simulink model "test_FAST_qLPVMPCflapIPC"  (R2023a)
settings: Solver=FixedStepAuto  StartTime=0.0  StopTime=OutTable.Time(end)  FixedStep=DT  RelTol=1e-3
values from neighbouring files (symbols this model uses):
  DT = 0.008    [initWorkspace.m]    (also in runCompareCtrl.m)
  ipcMaxRateCtrl = 13    [initWorkspace.m]
  ipcParCtrl = designMPC.ipcParCtrl    [initWorkspace.m]
  Lin_points : value not decoded    [DD_test.sldd]
undefined symbols (not defined in the file or in its folder): Rotor_Lambda
settings Model: DataDictionary=DD_test.sldd  ExtModeTrigMode=oneshot  Creator=Hazim Namik  LastModifiedBy=jdi
settings SolverCC: AlgebraicLoopSolver=TrustRegion  AutoInsertRateTranBlk=on
settings DataIOCC: LimitDataPoints=on  SaveFormat=Array  ReturnWorkspaceOutputs=off
settings OptimizationCC: BlockReduction=off  BooleanDataType=off  LifeSpan=inf
settings DebuggingCC: SaveWithParameterizedLinksMsg=none  UnderspecifiedInitializationDetection=Classic  MergeDetectMultiDrivingBlocksExec=none  SignalResolutionControl=TryResolveAllWithWarning  UnconnectedInputMsg=warning  UnconnectedOutputMsg=warning  UnconnectedLineMsg=warning  SFUnexpectedBacktrackingDiag=warning  SFNoUnconditionalDefaultTransitionDiag=warning  SFExecutionAtInitializationDiag=none  ArithmeticOperatorsInVariantConditions=warning
settings HardwareCC: ProdBitPerPointer=32  ProdBitPerSizeT=32  ProdBitPerPtrDiffT=32  ProdLargestAtomicFloat=None  ProdIntDivRoundTo=Undefined  ProdEndianess=Unspecified  ProdWordSize=32  ProdHWDeviceType=32-bit Generic  TargetUnknown=on
settings ModelReferenceCC: EnableRefExpFcnMdlSchedulingChecks=on  PropagateSignalLabelsOutOfModel=off
settings SFSimCC: SimUseLocalCustomCode=off  CustomCodeUndefinedFunction=UseInterfaceOnly
settings RTWCC: RTWUseLocalCustomCode=off  DLArmComputeVersion=19.05
settings CodeAppCC: StateflowObjectComments=on
settings GRTTargetCC: TargetLangStandard=C89/C90 (ANSI)
settings ConfigComp: CovMetricSettings=dw  CovSaveCumulativeToWorkspaceVar=on  CovSaveSingleToWorkspaceVar=on  CovExternalEMLEnable=off

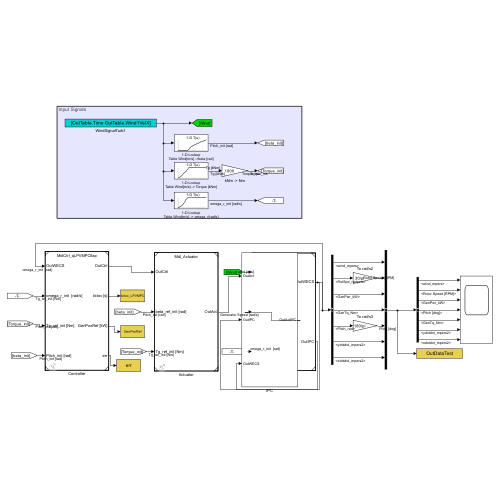
[thumbnail: Simulink's stored preview of the top-level diagram]
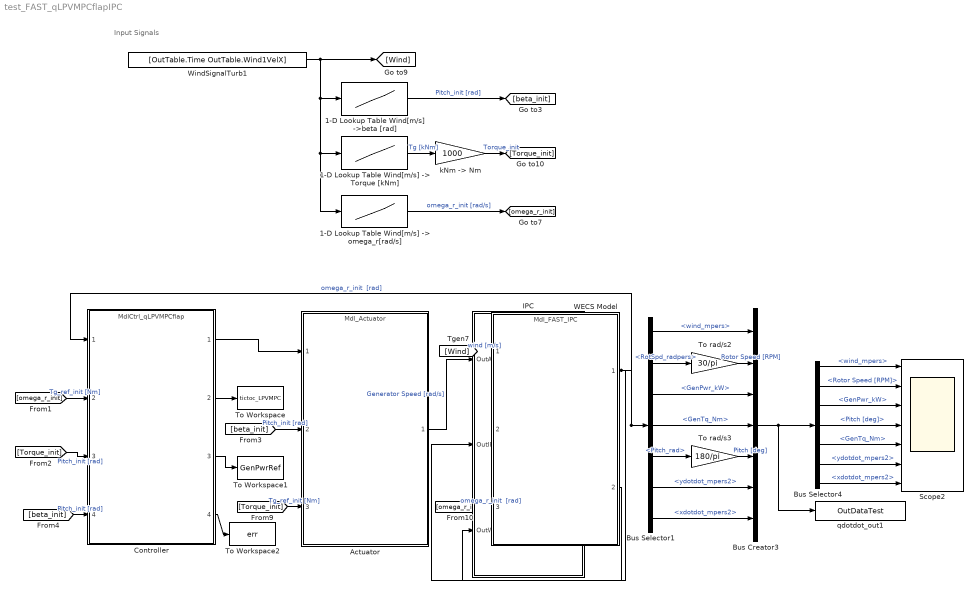
== system test_FAST_qLPVMPCflapIPC ==
  note: Input Signals
  "1-D Lookup Table Wind[m/s] -> Torque [kNm]" : Lookup_n-D  NumberOfTableDimensions=1  BreakpointsForDimension1=Lin_points.V  BreakpointsForDimension2=Rotor_Lambda  Table=Lin_points.Torque  InternalRulePriority=Speed  RndMeth=Simplest
  "1-D Lookup Table Wind[m/s] -> omega_r[rad/s]" : Lookup_n-D  NumberOfTableDimensions=1  BreakpointsForDimension1=Lin_points.V  BreakpointsForDimension2=Rotor_Lambda  Table=Lin_points.RSpeed  InternalRulePriority=Speed  RndMeth=Simplest
  1-D Lookup Table Wind[m/s] ->beta [rad] : Lookup_n-D  NumberOfTableDimensions=1  BreakpointsForDimension1=Lin_points.V  BreakpointsForDimension2=Rotor_Lambda  Table=Lin_points.Pitch  InternalRulePriority=Speed  RndMeth=Simplest
  Actuator : ModelReference  ModelNameDialog=Mdl_Actuator.slx  SimulationMode=Normal  ModelReferenceVersion=7.0
  Bus Creator3 : BusCreator  Inputs=7
  Bus Selector1 : BusSelector  OutputSignals=wind_mpers,RotSpd_radpers,GenPwr_kW,GenTq_Nm,Pitch_rad,ydotdot_mpers2,xdotdot_mpers2
  Bus Selector4 : BusSelector  OutputSignals=wind_mpers,Rotor Speed [RPM],GenPwr_kW,Pitch [deg],GenTq_Nm,ydotdot_mpers2,xdotdot_mpers2
  Controller : ModelReference  ModelNameDialog=MdlCtrl_qLPVMPCflap  SimulationMode=Normal  ModelReferenceVersion=7.57
  IPC : Subsystem
  Scope2 : Scope  NumInputPorts=7
      settings: Tag=Scope
  To Workspace : ToWorkspace  VariableName=tictoc_LPVMPC  SaveFormat=Timeseries  SampleTime=-1
  To Workspace1 : ToWorkspace  VariableName=GenPwrRef  SaveFormat=Timeseries  SampleTime=-1
  To Workspace2 : ToWorkspace  VariableName=err  SaveFormat=Timeseries  SampleTime=-1
  To rad/s2 : Gain  Gain=30/pi
  To rad/s3 : Gain  Gain=180/pi
  WECS Model : ModelReference  ModelNameDialog=Mdl_FAST_IPC  SimulationMode=Normal  ModelReferenceVersion=8.1
  WindSignalTurb1 : FromWorkspace  VariableName=[OutTable.Time OutTable.Wind1VelX]  SampleTime=DT  OutputAfterFinalValue=Holding final value
  "kNm -> Nm" : Gain  Gain=1000
  qdotdot_out1 : ToWorkspace  VariableName=OutDataTest  SampleTime=-1
  wires:
  [Torque_init] -> Controller/3  "Pitch_init [rad]"
  WindSignalTurb1/1 -> [Wind], "1-D Lookup Table Wind[m/s] -> omega_r[rad/s]"/1, "1-D Lookup Table Wind[m/s] -> Torque [kNm]"/1, 1-D Lookup Table Wind[m/s] ->beta [rad]/1
  "kNm -> Nm"/1 -> [Torque_init]  "Torque_init"
  [omega_r_init] -> Controller/2  "Tg_ref_init [Nm]"
  "1-D Lookup Table Wind[m/s] -> omega_r[rad/s]"/1 -> [omega_r_init]  "omega_r_init [rad/s]"
  [Wind] -> WECS Model/1  "wind [m/s]"
  1-D Lookup Table Wind[m/s] ->beta [rad]/1 -> [beta_init]  "Pitch_init [rad]"
  "1-D Lookup Table Wind[m/s] -> Torque [kNm]"/1 -> "kNm -> Nm"/1  "Tg [kNm]"
  [Torque_init] -> Actuator/3  "Tg_ref_init [Nm]"
  [omega_r_init] -> WECS Model/3  "omega_r_init  [rad]"
  Controller/3 -> To Workspace1/1
  [beta_init] -> Actuator/2  "Pitch_init [rad]"
  Bus Selector1/5 -> To rad/s3/1  "<Pitch_rad>"
  To rad/s2/1 -> Bus Creator3/2  "Rotor Speed [RPM]"
  Bus Creator3/1 -> Bus Selector4/1, qdotdot_out1/1
  Bus Selector4/4 -> Scope2/4  "<Pitch [deg]>"
  Bus Selector4/7 -> Scope2/7  "<xdotdot_mpers2>"
  Bus Selector4/6 -> Scope2/6  "<ydotdot_mpers2>"
  Bus Selector4/1 -> Scope2/1  "<wind_mpers>"
  To rad/s3/1 -> Bus Creator3/5  "Pitch [deg]"
  Bus Selector4/5 -> Scope2/5  "<GenTq_Nm>"
  Bus Selector1/2 -> To rad/s2/1  "<RotSpd_radpers>"
  Bus Selector1/1 -> Bus Creator3/1  "<wind_mpers>"
  Bus Selector1/4 -> Bus Creator3/4  "<GenTq_Nm>"
  Bus Selector1/3 -> Bus Creator3/3  "<GenPwr_kW>"
  Bus Selector1/7 -> Bus Creator3/7  "<xdotdot_mpers2>"
  Bus Selector1/6 -> Bus Creator3/6  "<ydotdot_mpers2>"
  Bus Selector4/3 -> Scope2/3  "<GenPwr_kW>"
  Bus Selector4/2 -> Scope2/2  "<Rotor Speed [RPM]>"
  WECS Model/1 -> Bus Selector1/1, Controller/1, IPC/3(OutWECS)  "omega_r_init  [rad]"
  [beta_init] -> Controller/4  "Pitch_init [rad]"
  Controller/1 -> Actuator/1
  Controller/2 -> To Workspace/1
  Controller/4 -> To Workspace2/1
  Actuator/1 -> IPC/1(OutAct)  "Generator Speed [rad/s]"
  WECS Model/2 -> IPC/2(OutIPC)
  IPC/1(OutActIPC) -> WECS Model/2

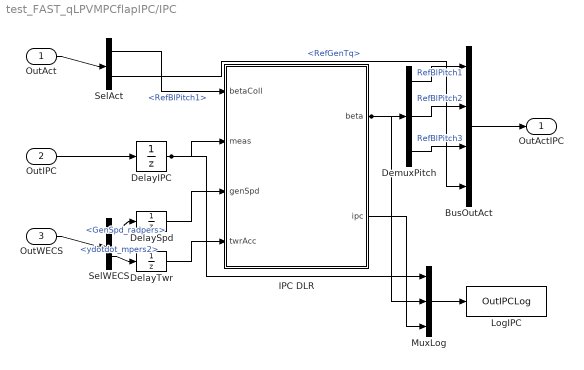
== system test_FAST_qLPVMPCflapIPC/IPC ==
  OutAct : Inport
  OutIPC : Inport  Port=2
  OutWECS : Inport  Port=3
  BusOutAct : BusCreator  Inputs=4
  DelayIPC : UnitDelay  InitialCondition=[0 0 0 0]  SampleTime=DT  HasFrameUpgradeWarning=on
  DelaySpd : UnitDelay  SampleTime=DT  HasFrameUpgradeWarning=on
  DelayTwr : UnitDelay  SampleTime=DT  HasFrameUpgradeWarning=on
  DemuxPitch : Demux  Outputs=3
  IPC DLR : MATLAB Function  TreatAsAtomicUnit=on
  LogIPC : ToWorkspace  VariableName=OutIPCLog  SampleTime=DT
  MuxLog : Mux  Inputs=3
  SelAct : BusSelector  OutputSignals=RefBlPitch1,RefGenTq
  SelWECS : BusSelector  OutputSignals=GenSpd_radpers,ydotdot_mpers2
  OutActIPC : Outport
  wires:
  OutAct/1 -> SelAct/1
  OutIPC/1 -> DelayIPC/1
  OutWECS/1 -> SelWECS/1
  SelWECS/1 -> DelaySpd/1  "<GenSpd_radpers>"
  SelWECS/2 -> DelayTwr/1  "<ydotdot_mpers2>"
  SelAct/1 -> IPC DLR/1(betaColl)  "<RefBlPitch1>"
  DelayIPC/1 -> IPC DLR/2(meas), MuxLog/1
  DelaySpd/1 -> IPC DLR/3(genSpd)
  DelayTwr/1 -> IPC DLR/4(twrAcc)
  IPC DLR/1(beta) -> DemuxPitch/1, MuxLog/2
  DemuxPitch/1 -> BusOutAct/1  "RefBlPitch1"
  DemuxPitch/2 -> BusOutAct/2  "RefBlPitch2"
  DemuxPitch/3 -> BusOutAct/3  "RefBlPitch3"
  SelAct/2 -> BusOutAct/4  "<RefGenTq>"
  BusOutAct/1 -> OutActIPC/1
  IPC DLR/2(ipc) -> MuxLog/3
  MuxLog/1 -> LogIPC/1

== matlab function test_FAST_qLPVMPCflapIPC/IPC/IPC DLR ==
  settings: updateMethod=DISCRETE  sampleTime=DT
  data: betaColl input; beta output; meas input; genSpd input; twrAcc input; ipc output; ipcParCtrl parameter; DT parameter; ipcMaxRateCtrl parameter
function [beta, ipc] = ipc_block(betaColl, meas, genSpd, twrAcc, ipcParCtrl, DT, ipcMaxRateCtrl)
% Individual pitch control on top of the collective pitch reference
% (ipc_dlr); meas = [RootMOoP1..3 (kNm), Azimuth (deg)], one sample delayed; ipcParCtrl = [gainSet, kScale, towerOn]
[beta, ipc] = ipc_dlr(betaColl, meas(1:3), meas(4), genSpd, twrAcc, ipcParCtrl, DT, ipcMaxRateCtrl);
